simulink model "GuidanceLaw"  (R2023b)
settings: Solver=ode4  StartTime=0.0  StopTime=400  FixedStep=0.05  RelTol=1e-3
values from neighbouring files (symbols this model uses):
  APCMD_TYPE : value not decoded    [apDataDictionary.sldd]
  missionRoutePlan_struct = struct(      'validWpNum_u8', uint8(5),      'missionRoute_struct', repmat(wpDefault_struct, double(maxWpNum_u8), 1))    [initMissionRoutePlan_MC.m]
  MSSN_TYPE : value not decoded    [apDataDictionary.sldd]
  setPoint_struct = struct('lat_deg_d',double(31.200000),'lon_deg_d',double(121.500000),'alt_m_f',single(100),'yaw_deg_f',single(0))    [APTest.m]
undefined symbols (not defined in the file or in its folder): apParams
libraries: simulink x13, simulink_extras x3
(part 7 of 7)

== matlab function GuidanceLaw/Subsystem/wpMssnHandle/WaypointArrivalState/cirJudge/MATLAB Function1 ==
  data: curPosNE_m_f input; cirJudge_b output; curWpNE_m_f input; nextWpNE_m_f input; cirExitTolerance_deg_f input; reset_b input
function cirJudge_b = cirJudge(curPosNE_m_f, curWpNE_m_f, nextWpNE_m_f, cirExitTolerance_deg_f, reset_b)
%#codegen
%
% 圆弧航点无附加条件到达判定
%
% curWpNE_m_f：圆弧圆心
% nextWpNE_m_f：圆弧切出点
%
% 当前方位角与切出方位角的最小夹角小于给定容差时，
% 判定圆弧航点完成。完成状态保持到reset_b复位。

persistent completeState_b

pN_m_f = curPosNE_m_f(1) - curWpNE_m_f(1);
pE_m_f = curPosNE_m_f(2) - curWpNE_m_f(2);

exitN_m_f = nextWpNE_m_f(1) - curWpNE_m_f(1);
exitE_m_f = nextWpNE_m_f(2) - curWpNE_m_f(2);

curBearing_rad_f = atan2(pE_m_f, pN_m_f);
exitBearing_rad_f = atan2(exitE_m_f, exitN_m_f);

angleErr_rad_f = atan2(sin(curBearing_rad_f - exitBearing_rad_f), cos(curBearing_rad_f - exitBearing_rad_f));

angleTolerance_rad_f = cirExitTolerance_deg_f * single(pi / 180.0);

if isempty(completeState_b)
    completeState_b = false;
end

if reset_b
    completeState_b = false;
elseif abs(angleErr_rad_f) < angleTolerance_rad_f
    completeState_b = true;
end

cirJudge_b = completeState_b;
end

== matlab function GuidanceLaw/MATLAB Function ==
  data: apCmd_struct input; nav_struct output Bus: apTransNavBus; dt_s_f input; initState_f input; refLat_deg_d input; refLon_deg_d input; refAlt_m_f input; groundAlt_m_f input; flightPhase_u8 output
function [nav_struct, flightPhase_u8] = simple6DofPlant(apCmd_struct, dt_s_f, initState_f, refLat_deg_d, refLon_deg_d, refAlt_m_f, groundAlt_m_f)
%#codegen
%
% 面向AP逻辑和功能验证的简化六自由度运动学模型。
%
% 设计原则：
% 1. 直接使用AP已经完成限幅、限速处理的速度和姿态指令；
% 2. 不再增加速度、加速度、jerk和姿态响应参数；
% 3. 旋翼阶段直接跟踪机体系速度、垂速和姿态角指令；
% 4. 倾转/固定翼阶段仅保留滚转角产生协调转弯这一必要运动学关系；
% 5. 飞行阶段根据离地高度和水平速度自动判定；
% 6. 输出字段与AP_v8(3)中的apTransNavBus完全一致；
% 7. 本拍输出当前状态，再用当前指令更新下一拍状态，避免直接馈通代数环。
%
% flightPhase_u8：
% 0 INVALID，1 MC_GROUND，2 MC_FLIGHT，3 TILT_FLIGHT，4 FW_FLIGHT。
%
% initState_f，12x1：
% 1:3   局部NEU位置[N;E;U]，m；
% 4:6   NEU速度[Vn;Ve;Vu]，m/s；
% 7:9   姿态角[roll;pitch;yaw]，deg；
% 10:12 机体系角速度[p;q;r]，deg/s。

persistent posStateNEU_m_f
persistent velStateNEU_mps_f
persistent accStateNEU_mps2_f
persistent attState_deg_f
persistent rateState_dps_f
persistent flightPhaseState_u8

if isempty(posStateNEU_m_f)
    posStateNEU_m_f = single(initState_f(1:3));
    velStateNEU_mps_f = single(initState_f(4:6));
    accStateNEU_mps2_f = single(zeros(3, 1));
    attState_deg_f = single(initState_f(7:9));
    attState_deg_f(3) = wrap180Single(attState_deg_f(3));
    rateState_dps_f = single(initState_f(10:12));
    flightPhaseState_u8 = initialFlightPhase(posStateNEU_m_f, velStateNEU_mps_f, refAlt_m_f, groundAlt_m_f);
end

%% 输出当前状态

posNEU_m_f = posStateNEU_m_f;
velNEU_mps_f = velStateNEU_mps_f;
accNEU_mps2_f = accStateNEU_mps2_f;
attEuler_deg_f = attState_deg_f;
rateBody_dps_f = rateState_dps_f;
flightPhase_u8 = flightPhaseState_u8;

nav_struct = makeNavOutput(posStateNEU_m_f, velStateNEU_mps_f, accStateNEU_mps2_f, attState_deg_f, rateState_dps_f, refLat_deg_d, refLon_deg_d, refAlt_m_f, groundAlt_m_f);

% AP未运行时保持当前状态，清除运动学导数。
if ~logical(apCmd_struct.apRunState_b)
    accStateNEU_mps2_f = single(zeros(3, 1));
    rateState_dps_f = single(zeros(3, 1));
    return;
end

%% 基本常量

dtUse_s_f = max(single(dt_s_f), single(0.0001));

DEG2RAD_F = single(pi / 180.0);
RAD2DEG_F = single(180.0 / pi);
GRAVITY_MPS2_F = single(9.80665);
MIN_TURN_SPD_MPS_F = single(1.0);

isMcPhase_b = flightPhaseState_u8 == uint8(1) || flightPhaseState_u8 == uint8(2);

%% 姿态更新

attNext_deg_f = attState_deg_f;
attNext_deg_f(1) = single(apCmd_struct.rollCmd_deg_f);
attNext_deg_f(2) = single(apCmd_struct.pitchCmd_deg_f);

if isMcPhase_b
    attNext_deg_f(3) = wrap180Single(single(apCmd_struct.yawCmd_deg_f));
else
    tasCmd_mps_f = max(single(apCmd_struct.vxCmd_mps_f), single(0.0));
    yawRate_dps_f = single(0.0);

    if tasCmd_mps_f > MIN_TURN_SPD_MPS_F
        rollCmd_rad_f = attNext_deg_f(1) * DEG2RAD_F;
        yawRate_dps_f = GRAVITY_MPS2_F * tan(rollCmd_rad_f) / tasCmd_mps_f * RAD2DEG_F;
    end

    attNext_deg_f(3) = wrap180Single(attState_deg_f(3) + yawRate_dps_f * dtUse_s_f);
end

%% 速度更新

yawNext_rad_f = attNext_deg_f(3) * DEG2RAD_F;
cosYaw_f = cos(yawNext_rad_f);
sinYaw_f = sin(yawNext_rad_f);

velNextNEU_mps_f = single(zeros(3, 1));

if isMcPhase_b
    vxCmd_mps_f = single(apCmd_struct.vxCmd_mps_f);
    vyCmd_mps_f = single(apCmd_struct.vyCmd_mps_f);

    velNextNEU_mps_f(1) = cosYaw_f * vxCmd_mps_f - sinYaw_f * vyCmd_mps_f;
    velNextNEU_mps_f(2) = sinYaw_f * vxCmd_mps_f + cosYaw_f * vyCmd_mps_f;
    velNextNEU_mps_f(3) = single(apCmd_struct.vuCmd_mps_f);
else
    tasCmd_mps_f = max(single(apCmd_struct.vxCmd_mps_f), single(0.0));
    vuCmd_mps_f = single(apCmd_struct.vuCmd_mps_f);
    horizonSpdCmd_mps_f = sqrt(max(tasCmd_mps_f * tasCmd_mps_f - vuCmd_mps_f * vuCmd_mps_f, single(0.0)));

    velNextNEU_mps_f(1) = horizonSpdCmd_mps_f * cosYaw_f;
    velNextNEU_mps_f(2) = horizonSpdCmd_mps_f * sinYaw_f;
    velNextNEU_mps_f(3) = vuCmd_mps_f;
end

%% 由相邻状态计算加速度和机体系角速度

accNextNEU_mps2_f = (velNextNEU_mps_f - velStateNEU_mps_f) / dtUse_s_f;

eulerRate_dps_f = single(zeros(3, 1));
eulerRate_dps_f(1) = (attNext_deg_f(1) - attState_deg_f(1)) / dtUse_s_f;
eulerRate_dps_f(2) = (attNext_deg_f(2) - attState_deg_f(2)) / dtUse_s_f;
eulerRate_dps_f(3) = wrap180Single(attNext_deg_f(3) - attState_deg_f(3)) / dtUse_s_f;

roll_rad_f = attState_deg_f(1) * DEG2RAD_F;
pitch_rad_f = attState_deg_f(2) * DEG2RAD_F;

rateNext_dps_f = single(zeros(3, 1));
rateNext_dps_f(1) = eulerRate_dps_f(1) - eulerRate_dps_f(3) * sin(pitch_rad_f);
rateNext_dps_f(2) = eulerRate_dps_f(2) * cos(roll_rad_f) + eulerRate_dps_f(3) * sin(roll_rad_f) * cos(pitch_rad_f);
rateNext_dps_f(3) = -eulerRate_dps_f(2) * sin(roll_rad_f) + eulerRate_dps_f(3) * cos(roll_rad_f) * cos(pitch_rad_f);

%% 位置积分和地面约束

posNextNEU_m_f = posStateNEU_m_f + single(0.5) * (velStateNEU_mps_f + velNextNEU_mps_f) * dtUse_s_f;

altNext_m_f = single(refAlt_m_f) + posNextNEU_m_f(3);

if altNext_m_f < single(groundAlt_m_f)
    posNextNEU_m_f(3) = single(groundAlt_m_f) - single(refAlt_m_f);

    if velNextNEU_mps_f(3) < single(0.0)
        velNextNEU_mps_f(3) = single(0.0);
        accNextNEU_mps2_f(3) = single(0.0);
    end
end

%% 自动更新飞行阶段

flightPhaseNext_u8 = updateFlightPhase(flightPhaseState_u8, posNextNEU_m_f, velNextNEU_mps_f, refAlt_m_f, groundAlt_m_f);

%% 保存下一拍状态

posStateNEU_m_f = posNextNEU_m_f;
velStateNEU_mps_f = velNextNEU_mps_f;
accStateNEU_mps2_f = accNextNEU_mps2_f;
attState_deg_f = attNext_deg_f;
rateState_dps_f = rateNext_dps_f;
flightPhaseState_u8 = flightPhaseNext_u8;

end


function flightPhase_u8 = initialFlightPhase(posNEU_m_f, velNEU_mps_f, refAlt_m_f, groundAlt_m_f)
%#codegen

hag_m_f = single(refAlt_m_f) + posNEU_m_f(3) - single(groundAlt_m_f);
horizonSpd_mps_f = single(hypot(double(velNEU_mps_f(1)), double(velNEU_mps_f(2))));

if hag_m_f <= single(0.1)
    flightPhase_u8 = uint8(1);
elseif horizonSpd_mps_f < single(12.0)
    flightPhase_u8 = uint8(2);
elseif horizonSpd_mps_f < single(30.0)
    flightPhase_u8 = uint8(3);
else
    flightPhase_u8 = uint8(4);
end

end


function flightPhaseNext_u8 = updateFlightPhase(flightPhase_u8, posNEU_m_f, velNEU_mps_f, refAlt_m_f, groundAlt_m_f)
%#codegen
%
% 简化飞行阶段判定，带速度和高度滞环：
% MC_GROUND -> MC_FLIGHT：HAG > 0.3 m；
% MC_FLIGHT -> TILT_FLIGHT：水平速度 >= 12 m/s；
% TILT_FLIGHT -> MC_FLIGHT：水平速度 <= 10 m/s；
% TILT_FLIGHT -> FW_FLIGHT：水平速度 >= 30 m/s；
% FW_FLIGHT -> TILT_FLIGHT：水平速度 <= 28 m/s；
% 任意空中阶段 -> MC_GROUND：HAG <= 0.1 m。

hag_m_f = single(refAlt_m_f) + posNEU_m_f(3) - single(groundAlt_m_f);
horizonSpd_mps_f = single(hypot(double(velNEU_mps_f(1)), double(velNEU_mps_f(2))));

flightPhaseNext_u8 = flightPhase_u8;

switch flightPhase_u8
    case uint8(1)
        if hag_m_f > single(0.3)
            flightPhaseNext_u8 = uint8(2);
        end

    case uint8(2)
        if hag_m_f <= single(0.1)
            flightPhaseNext_u8 = uint8(1);
        elseif horizonSpd_mps_f >= single(12.0)
            flightPhaseNext_u8 = uint8(3);
        end

    case uint8(3)
        if hag_m_f <= single(0.1)
            flightPhaseNext_u8 = uint8(1);
        elseif horizonSpd_mps_f >= single(30.0)
            flightPhaseNext_u8 = uint8(4);
        elseif horizonSpd_mps_f <= single(10.0)
            flightPhaseNext_u8 = uint8(2);
        end

    case uint8(4)
        if hag_m_f <= single(0.1)
            flightPhaseNext_u8 = uint8(1);
        elseif horizonSpd_mps_f <= single(28.0)
            flightPhaseNext_u8 = uint8(3);
        end

    otherwise
        flightPhaseNext_u8 = initialFlightPhase(posNEU_m_f, velNEU_mps_f, refAlt_m_f, groundAlt_m_f);
end

end


function nav_struct = makeNavOutput(posNEU_m_f, velNEU_mps_f, accNEU_mps2_f, att_deg_f, rate_dps_f, refLat_deg_d, refLon_deg_d, refAlt_m_f, groundAlt_m_f)
%#codegen

EARTH_RADIUS_M_D = 6371000.0;
RAD2DEG_D = 180.0 / pi;

lat_deg_d = double(refLat_deg_d) + double(posNEU_m_f(1)) / EARTH_RADIUS_M_D * RAD2DEG_D;
longitudeScale_d = max(cos(double(refLat_deg_d) * pi / 180.0), 0.01);
lon_deg_d = double(refLon_deg_d) + double(posNEU_m_f(2)) / (EARTH_RADIUS_M_D * longitudeScale_d) * RAD2DEG_D;
lon_deg_d = mod(lon_deg_d + 180.0, 360.0) - 180.0;

alt_m_f = single(refAlt_m_f) + posNEU_m_f(3);
hag_m_f = max(alt_m_f - single(groundAlt_m_f), single(0.0));
vg_mps_f = single(hypot(double(velNEU_mps_f(1)), double(velNEU_mps_f(2))));
tas_mps_f = single(sqrt(double(velNEU_mps_f(1) * velNEU_mps_f(1) + velNEU_mps_f(2) * velNEU_mps_f(2) + velNEU_mps_f(3) * velNEU_mps_f(3))));

nav_struct = struct('lat_deg_d', lat_deg_d, 'lon_deg_d', lon_deg_d, 'lonlatValid_b', true, 'alt_m_f', alt_m_f, 'altValid_b', true, 'velN_mps_f', velNEU_mps_f(1), 'velE_mps_f', velNEU_mps_f(2), 'velNEValid_b', true, 'velU_mps_f', velNEU_mps_f(3), 'velUValid_b', true, 'accN_mps2_f', accNEU_mps2_f(1), 'accE_mps2_f', accNEU_mps2_f(2), 'accU_mps2_f', accNEU_mps2_f(3), 'roll_deg_f', att_deg_f(1), 'pitch_deg_f', att_deg_f(2), 'attValid_b', true, 'yaw_deg_f', wrap180Single(att_deg_f(3)), 'yawValid_b', true, 'p_dps_f', rate_dps_f(1), 'q_dps_f', rate_dps_f(2), 'r_dps_f', rate_dps_f(3), 'hag_m_f', hag_m_f, 'hagValid_b', true, 'vg_mps_f', vg_mps_f, 'vgValid_b', true, 'tas_mps_f', tas_mps_f, 'tasValid_b', true);

end


function angle_deg_f = wrap180Single(angle_deg_f)
%#codegen

angle_deg_f = mod(angle_deg_f + single(180.0), single(360.0)) - single(180.0);

end

== matlab function GuidanceLaw/MATLAB Function1 ==
  data: simTime_s_d input; apTaskCmd_enum output
function apTaskCmd_enum = apTaskCmdPulse(simTime_s_d)
%#codegen
%
% 1.00~1.10 s触发垂直起飞，其余时间为无效指令

apTaskCmd_enum = AP_TASK_CMD.INVALID_CMD;

if simTime_s_d >= 1.0 && simTime_s_d < 1.1
    apTaskCmd_enum = AP_TASK_CMD.VERTICAL_TAKEOFF_CMD;
end

% if simTime_s_d >= 100.0 && simTime_s_d < 100.1
%     apTaskCmd_enum = AP_TASK_CMD.RTH_CMD;
% end

end

== matlab function GuidanceLaw/Subsystem/wpMssnHandle/GuiLaw/yawGuidance/yawCmdLimit/cldWrap180 ==
  data: u input; y output
function y = fcn(u)
    y = cldWrap180(u);
end

== matlab function GuidanceLaw/Subsystem/wpMssnHandle/GuiLaw/yawGuidance/yawCmdLimit/cldWrap1801 ==
  data: u input; y output
function y = fcn(u)
    y = cldWrap180(u);
end

== matlab function GuidanceLaw/Subsystem/wpMssnHandle/WaypointArrivalState/mcLineJudge/JudgeAlgorithm1 ==
  data: curPosNE_m_f input; mcLineJudge_b output; preWpNE_m_f input; curWpNE_m_f input; nextWpNE_m_f input; targetTurnSpeed_mps_f input; maxLatAcc_mps2_f input; minJudgeDist_m_f input; maxJudgeDist_m_f input; segmentLimitRatio_f input; reset_b input
function mcLineJudge_b = mcLineJudge(curPosNE_m_f, preWpNE_m_f, curWpNE_m_f, nextWpNE_m_f, targetTurnSpeed_mps_f, maxLatAcc_mps2_f, ...
    minJudgeDist_m_f, maxJudgeDist_m_f, segmentLimitRatio_f, reset_b)
%#codegen
%
% 旋翼直线航点提前分界面判定
%
% geometryState_f：
% 1  提前判定距离，m
% 2  A->B单位方向北向分量
% 3  A->B单位方向东向分量
% 4  B点在A->B单位方向上的投影，m

persistent completeState_b
persistent geometryState_f
persistent init_b

smallValue_m_f = single(0.001);
zero_f = single(0.0);
one_f = single(1.0);

%% 状态初始化

% 每个持久变量必须分别检查和初始化
if isempty(init_b)
    completeState_b = false;
    geometryState_f = single(zeros(4, 1));
    init_b = true;
end

%% 新航段几何计算与冻结
if init_b || reset_b
    completeState_b = false;
    geometryState_f = single(zeros(4, 1));
    init_b = false;

    % 当前航段A->B和下一航段B->C的水平向量。
    inN_m_f = curWpNE_m_f(1) - preWpNE_m_f(1);
    inE_m_f = curWpNE_m_f(2) - preWpNE_m_f(2);
    outN_m_f = nextWpNE_m_f(1) - curWpNE_m_f(1);
    outE_m_f = nextWpNE_m_f(2) - curWpNE_m_f(2);

    inLength_m_f = sqrt(inN_m_f * inN_m_f + inE_m_f * inE_m_f);
    outLength_m_f = sqrt(outN_m_f * outN_m_f + outE_m_f * outE_m_f);

    minDist_m_f = max(minJudgeDist_m_f, zero_f);
    maxDist_m_f = max(maxJudgeDist_m_f, minDist_m_f);
    segmentRatio_f = min(max(segmentLimitRatio_f, zero_f), single(0.49));

    % 小于该距离的当前航段直接完成。
    shortLineThreshold_m_f = max(minDist_m_f, smallValue_m_f);

    if inLength_m_f <= shortLineThreshold_m_f
        % 当前航段A->B过短，无须继续执行分界面判定。
        completeState_b = true;
        
    else
        % 当前航段有效，计算并冻结A->B方向。
        inDirN_f = inN_m_f / inLength_m_f;
        inDirE_f = inE_m_f / inLength_m_f;

        judgeDist_m_f = zero_f;
        judgeGeometryReady_b = false;

        if outLength_m_f <= shortLineThreshold_m_f
            % 下一航段过短，无法计算有效转角。
            % 当前航段退化为按最小提前距离进行判定。
            geometryMaxDist_m_f = segmentRatio_f * inLength_m_f;
            effectiveMaxDist_m_f = min(maxDist_m_f, geometryMaxDist_m_f);
            judgeDist_m_f = min(minDist_m_f, effectiveMaxDist_m_f);
            judgeGeometryReady_b = true;

        else
            outDirN_f = outN_m_f / outLength_m_f;
            outDirE_f = outE_m_f / outLength_m_f;

            % 计算A->B与B->C之间的水平转角。
            turnCos_f = inDirN_f * outDirN_f + inDirE_f * outDirE_f;
            turnCos_f = min(max(turnCos_f, -one_f), one_f);
            turnAngle_rad_f = acos(turnCos_f);

            % 根据R=v^2/a计算转弯半径。
            turnRadius_m_f = zero_f;

            if abs(targetTurnSpeed_mps_f) > smallValue_m_f && maxLatAcc_mps2_f > smallValue_m_f
                turnRadius_m_f = targetTurnSpeed_mps_f * targetTurnSpeed_mps_f / maxLatAcc_mps2_f;
            end

            if turnRadius_m_f > smallValue_m_f
                % 根据L=R*tan(turnAngle/2)计算理论提前距离。
                halfTurnAngle_rad_f = min(single(0.5) * turnAngle_rad_f, single(89.0 * pi / 180.0));
                rawJudgeDist_m_f = turnRadius_m_f * tan(halfTurnAngle_rad_f);

                % 提前距离受参数和相邻航段长度共同限制。
                geometryMaxDist_m_f = segmentRatio_f * min(inLength_m_f, outLength_m_f);
                effectiveMaxDist_m_f = min(maxDist_m_f, geometryMaxDist_m_f);

                if effectiveMaxDist_m_f >= minDist_m_f
                    judgeDist_m_f = min(max(rawJudgeDist_m_f, minDist_m_f), effectiveMaxDist_m_f);
                else
                    judgeDist_m_f = effectiveMaxDist_m_f;
                end

                judgeGeometryReady_b = true;
            end
        end

        if judgeGeometryReady_b
            % 冻结当前航段分界面判定所需参数。
            geometryState_f(1) = judgeDist_m_f;
            geometryState_f(2) = inDirN_f;
            geometryState_f(3) = inDirE_f;
            geometryState_f(4) = curWpNE_m_f(1) * inDirN_f + curWpNE_m_f(2) * inDirE_f;
        end
    end
end

%% 提取冻结参数
judgeDist_m_f = geometryState_f(1);
inDirN_f = geometryState_f(2);
inDirE_f = geometryState_f(3);
curWpAlong_m_f = geometryState_f(4);

%% 提前分界面判定
% reset_b触发周期已经完成新航段初始化，本周期继续使用新航段几何参数进行判定。
if ~completeState_b
    curPosAlong_m_f = curPosNE_m_f(1) * inDirN_f + curPosNE_m_f(2) * inDirE_f;
    remainDist_m_f = curWpAlong_m_f - curPosAlong_m_f;

    if remainDist_m_f <= judgeDist_m_f
        completeState_b = true;
    end
end

% 完成后保持到下一次segSwitch_b触发。
mcLineJudge_b = completeState_b;

end
